simulink model "cp6_ej1_smith"  (R2026a)
settings: Solver=VariableStepAuto  StopTime=20  MaxStep=0.002
libraries: slpidlib x1
settings Model: Creator=benja  LastModifiedBy=benja

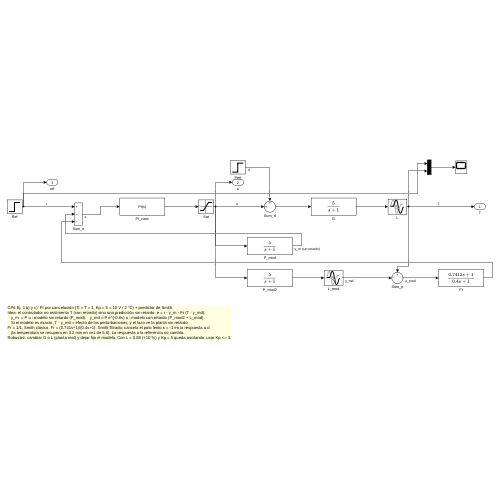
[thumbnail: Simulink's stored preview of the top-level diagram]
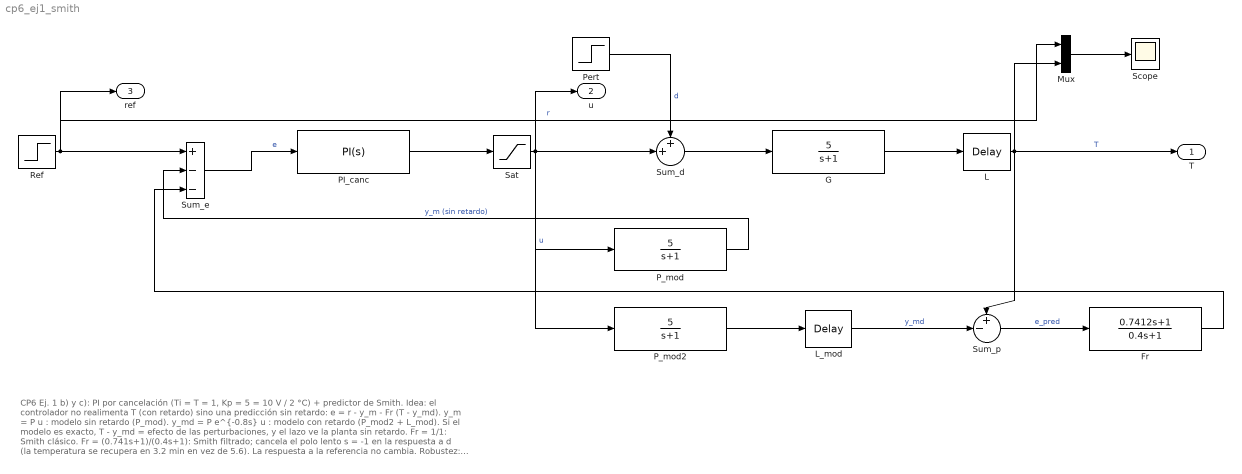
== system cp6_ej1_smith ==
  note: CP6 Ej. 1 b) y c): PI por cancelación (Ti = T = 1, Kp = 5 = 10 V / 2 °C) + predictor de Smith.
      | Idea: el controlador no realimenta T (con retardo) sino una predicción sin retardo: e = r - y_m - Fr (T - y_md).
      |    y_m  = P u : modelo sin retardo (P_mod).   y_md = P e^{-0.8s} u : modelo con retardo (P_mod2 + L_mod).
      |    Si el modelo es exacto, T - y_md = efecto de las perturbaciones, y el lazo ve la planta sin retardo.
      | Fr = 1/1: Smith clásico. Fr = (0.741s+1)/(0.4s+1): Smith filtrado; cancela el polo lento s = -1 en la respuesta a d
      |    (la temperatura se recupera en 3.2 min en vez de 5.6). La respuesta a la referencia no cambia.
      | Robustez: cambiar G o L (planta real) y dejar fijo el modelo. Con L = 0.88 (+10 %) y Kp = 5 queda oscilando: usar Kp <= 3.
  Fr : TransferFcn  Numerator=[0.7412 1]  Denominator=[0.4 1]
  G : TransferFcn  Numerator=5  Denominator=[1 1]
  L : TransportDelay  DelayTime=0.8
  L_mod : TransportDelay  DelayTime=0.8
  Mux : Mux  Inputs=2
  PI_canc : slpidlib/PID Controller  Controller=PI  Form=Parallel  TimeDomain=Continuous-time  UseExternalTs=off  SampleTime=-1  IntegratorMethod=Forward Euler  FilterMethod=Forward Euler  ControllerParametersSource=internal  P=5  I=5  UseKiTs=off  D=0  UseExternalDerivativeSource=off  N=100  UseFilter=on  TunerSelectOption=Transfer Function Based (PID Tuner App)  InitialConditionSource=internal  InitialConditionForIntegrator=0  InitialConditionForFilter=0  DifferentiatorICPrevScaledInput=0  ExternalReset=none  TrackingMode=off  Kt=1  LimitOutput=off  SatLimitsSource=internal  UpperSaturationLimit=inf  LowerSaturationLimit=-inf  LinearizeAsGain=on  AntiWindupMode=none  Kb=1  LimitIntegrator=off  UpperIntegratorSaturationLimit=inf  LowerIntegratorSaturationLimit=-inf  POutMin=[]  POutMax=[]  IOutMin=[]  IOutMax=[]  DOutMin=[]  DOutMax=[]  NOutMin=[]  NOutMax=[]  SumOutMin=[]  SumOutMax=[]  SaturationOutMin=[]  SaturationOutMax=[]  PParamMin=[]  PParamMax=[]  IParamMin=[]  IParamMax=[]  DParamMin=[]  DParamMax=[]  NParamMin=[]  NParamMax=[]  KbParamMin=[]  KbParamMax=[]  KtParamMin=[]  KtParamMax=[]  KbOutMin=[]  KbOutMax=[]  KtOutMin=[]  KtOutMax=[]  IntegratorOutMin=[]  IntegratorOutMax=[]  FilterOutMin=[]  FilterOutMax=[]  SumI1OutMin=[]  SumI1OutMax=[]  SumI2OutMin=[]  SumI2OutMax=[]  SumI3OutMin=[]  SumI3OutMax=[]  SumI4OutMin=[]  SumI4OutMax=[]  SumDOutMin=[]  SumDOutMax=[]  DifferentiatorOutMin=[]  DifferentiatorOutMax=[]  FilterDiffOutCoefMin=[]  FilterDiffOutCoefMax=[]  ReciprocalOutMin=[]  ReciprocalOutMax=[]  SumDenOutMin=[]  SumDenOutMax=[]  SumNumOutMin=[]  SumNumOutMax=[]  DivideOutMin=[]  DivideOutMax=[]  UdiffTsProdOutMin=[]  UdiffTsProdOutMax=[]  NTsProdOutMin=[]  NTsProdOutMax=[]  UintegralTsProdOutMin=[]  UintegralTsProdOutMax=[]  UngainTsProdOutMin=[]  UngainTsProdOutMax=[]  ClampingZeroOutDataTypeStr=Inherit: Inherit via back propagation  ClampingZeroOutMin=[]  ClampingZeroOutMax=[]  FilterDenConstantOutDataTypeStr=Inherit: Inherit via back propagation  FilterDenConstantOutMin=[]  FilterDenConstantOutMax=[]  PCopyOutDataTypeStr=Inherit: Inherit via back propagation  PCopyOutMin=[]  PCopyOutMax=[]  NCopyOutDataTypeStr=Inherit: Inherit via back propagation  NCopyOutMin=[]  NCopyOutMax=[]  IntegratorContinuousStateAttributes=''  IntegratorStateMustResolveToSignalObject=off  IntegratorRTWStateStorageClass=Auto  FilterContinuousStateAttributes=''  FilterStateMustResolveToSignalObject=off  FilterRTWStateStorageClass=Auto  ParallelPVariant=InternalParameters  IdealPVariant=Disabled  IVariant=InternalParameters  DVariant=Disabled  IntegratorVariant=Continuous  SatVariant=Disabled  AWVariant=Passthrough  PCopyVariant=Disabled  TRVariant=Disabled  FdbkBlocksVariant=Forward  IdealPFdbkVariant=Disabled  SatFdbkVariant=Disabled  DerivativeFilterVariant=Disabled  NVariant=Disabled  NCopyVariant=Disabled_SignalSpec  FilterICVariant=Disabled  IntegratorICVariant=InternalICs  ExternalResetVariant=Disabled  TRSumVariant=Passthrough  SumFdbkVariant=Disabled  SumVariant=Sum_PI  TsampFilterVariant=InternalTs  TsampNgainVariant=Passthrough  TsampIntegralVariant=Disabled_SignalSpec  ExternalSaturationOutDataTypeStr=Inherit: Same as second input  DerivativeSourceVariant=Disabled  PreIntVariant=InternalPreInt
  P_mod : TransferFcn  Numerator=5  Denominator=[1 1]
  P_mod2 : TransferFcn  Numerator=5  Denominator=[1 1]
  Pert : Step  Time=10  FinalValue=0.1  SampleTime=0
  Ref : Step  FinalValue=2  SampleTime=0
  Sat : Saturate  UpperLimit=10  LowerLimit=0
  Scope : Scope
  Sum_d : Sum  Inputs=++|
  Sum_e : Sum  Inputs=+--
  Sum_p : Sum  Inputs=+-|
  T : Outport
  u : Outport  Port=2
  ref : Outport  Port=3
  wires:
  Ref/1 -> Sum_e/1, ref/1, Mux/1  "r"
  Sum_e/1 -> PI_canc/1  "e"
  PI_canc/1 -> Sat/1
  Sat/1 -> Sum_d/2, P_mod/1, P_mod2/1, u/1  "u"
  Pert/1 -> Sum_d/1  "d"
  Sum_d/1 -> G/1
  G/1 -> L/1
  L/1 -> T/1, Sum_p/1, Mux/2  "T"
  P_mod/1 -> Sum_e/2  "y_m (sin retardo)"
  P_mod2/1 -> L_mod/1
  L_mod/1 -> Sum_p/2  "y_md"
  Sum_p/1 -> Fr/1  "e_pred"
  Fr/1 -> Sum_e/3
  Mux/1 -> Scope/1
